simulink model "WaveStar"  (R2020b)
settings: Solver=ode8  StartTime=0  StopTime=225  FixedStep=0.05  MaxStep=0.05  RelTol=1e-3  EnableMultiTasking=on
values from neighbouring files (symbols this model uses):
  Ad = sysD.A    [controller_init.m]
  alpha_eff = ( eta_motoring + eta_generator ) / 2    (= 1.06428571429)    [controller_init.m]
  ARorder = 18    [controller_init.m]
  ARtrainingSet = 10    [controller_init.m]
  Bd = sysD.B    [controller_init.m]
  beta_eff = ( eta_motoring - eta_generator ) / 2    (= 0.364285714286)    [controller_init.m]
  dt = simu.dt    [controller_init.m]
  eta_generator = 0.7    [controller_init.m]
  eta_motoring = 1 / 0.7    (= 1.42857142857)    [controller_init.m]
  excM_precalculated = excM_stored    [controller_init.m]
  L_AB = 0.412    [controller_init.m]
  L_AC = 0.2    [controller_init.m]
  LAfloat = 0.54875    [controller_init.m]
  McSat = 12    [controller_init.m]
  Np = 40    [controller_init.m]
  phi_eff = 1000    [controller_init.m]
  predictionType = 2    [controller_init.m]
  prop_gain = 19.40;  load('waveData/SS6_excM_stored.mat')    [controller_init.m]
  Qkf = blkdiag( Qp, Qv, QradM, QexcM )    [controller_init.m]
  qnl = [ 0, 1; 1, 0 ]    [controller_init.m]
  R_ctrl = 0.90*eye( Np*nu )    [controller_init.m]
  Rkf = blkdiag( Rp, Rv )    [controller_init.m]
  startController = 15    [controller_init.m]
  startPredictor = 10    [controller_init.m]
  Theta0 = deg2rad(26.9527)    [controller_init.m]
  Umax = McSat    (= 12)    [controller_init.m]
  Umin = -McSat    (= -12)    [controller_init.m]
  xPcTs = dt    [controller_init.m]
undefined symbols (not defined in the file or in its folder): body, constraint, geometry, HPfreq, hydroData, LPfreq, pto, X, Y, Z
libraries: nesl_utility x9, WECSim_Lib_Constraints x5, WECSim_Lib_Body_Elements x5, sm_lib x5, WECSim_Lib_Frames x1
settings Model: Creator=kmruehl  LastModifiedBy=akeeste
settings SolverCC: ZeroCrossControl=DisableAll  AutoInsertRateTranBlk=on
settings DataIOCC: ReturnWorkspaceOutputs=off
settings OptimizationCC: LifeSpan=inf  SimCompilerOptimization=on
settings DebuggingCC: SFUnexpectedBacktrackingDiag=warning  SFNoUnconditionalDefaultTransitionDiag=warning  SFExecutionAtInitializationDiag=none  ArithmeticOperatorsInVariantConditions=warning
settings ModelReferenceCC: ModelReferenceMinAlgLoopOccurrences=on
settings SFSimCC: SimUseLocalCustomCode=off  CustomCodeUndefinedFunction=UseInterfaceOnly
settings RTWCC: RTWUseLocalCustomCode=off
settings CodeAppCC: StateflowObjectComments=on
settings GRTTargetCC: TargetLangStandard=C89/C90 (ANSI)
settings ConfigComp: CovMetricSettings=dw  CovSaveCumulativeToWorkspaceVar=on  CovSaveSingleToWorkspaceVar=on  CovExternalEMLEnable=off
settings SimscapeCC: SimscapeNormalizeSystem=off
settings ExplorerConfigSet: SimMechanicsOpenEditorOnUpdate=off  InternalSimMechanicsExplorerSettings="<ExplorerConfiguration><canonicalview>default</canonicalview><AnimationSetting><BasePlaybackSpeed>1.0</BasePlaybackSpeed><PlaybackSpeedFactor>1.0</PlaybackSpeedFactor></AnimationSetting><TilePanel><TileInfo><Tiles Columns=\"2\" Count=\"4\" Rows=\"2\"><Column Left=\"2\" Weight=\"0.4998\"/><Column Left=\"667\" Weight=\"0.5002\"/><Column Left=\"1333\"/><Row Top=\"2\" Weight=\"0.4997\"/><Row Top=\"952\" Weight=\"0.5003\"/><Row Top=\"1904\"/><Tile Height=\"1\" Width=\"1\" X=\"0\" Y=\"0\"/><Tile Height=\"1\" Width=\"1\" X=\"0\" Y=\"1\"/><Tile Height=\"1\" Width=\"1\" X=\"1\" Y=\"0\"/><Tile Height=\"1\" Width=\"1\" X=\"1\" Y=\"1\"/></Tiles></TileInfo><SceneInfo><SceneViewer><BGColor><R>0.60000002384185791</R><G>0.60000002384185791</G><B>0.60000002384185791</B></BGColor><Camera><DoPerspective>off</DoPerspective><Position><X>0.12470049519875293</X><Y>-7.8483064192972183</Y><Z>0.41049948909937695</Z></Position><Center><X>0.12470049519875293</X><Y>2.8810501090381635e-07</Y><Z>0.41049948909937695</Z></Center><Up><X>0</X><Y>-0</Y><Z>1</Z></Up><ViewLimDist>1</ViewLimDist><YLim>1.4359338132666335</YLim><XLim>1.0010335616396511</XLim></Camera></SceneViewer><SceneViewer><BGColor><R>0.60000002384185791</R><G>0.60000002384185791</G><B>0.60000002384185791</B></BGColor><Camera><DoPerspective>off</DoPerspective><Position><X>0.32732511337828807</X><Y>-0.082581165896399134</Y><Z>7.1171098135796953</Z></Position><Center><X>0.32732511337828807</X><Y>-0.082581165896399134</Y><Z>0.45174407037336595</Z></Center><Up><X>0</X><Y>1</Y><Z>-0</Z></Up><ViewLimDist>1</ViewLimDist><YLim>1.40160176353799</YLim><XLim>0.97502731376555829</XLim></Camera></SceneViewer><SceneViewer><BGColor><R>0.60000002384185791</R><G>0.60000002384185791</G><B>0.60000002384185791</B></BGColor><Camera><DoPerspective>off</DoPerspective><Position><X>7.848306419447999</X><Y>0.086028706913199554</Y><Z>0.42305679091343457</Z></Position><Center><X>-3.0318302890464111e-07</X><Y>0.086028706913199554</Y><Z>0.42305679091343457</Z></Center><Up><X>-0</X><Y>0</Y><Z>1</Z></Up><ViewLimDist>1</ViewLimDist><YLim>1.4671457032424258</YLim><XLim>1.0243514633690476</XLim></Camera></SceneViewer><SceneViewer><BGColor><R>0.60000002384185791</R><G>0.60000002384185791</G><B>0.60000002384185791</B></BGColor><Camera><DoPerspective>off</DoPerspective><Position><X>4.3109367218514292</X><Y>-3.7387044463777657</Y><Z>4.7725637716535374</Z></Position><Center><X>-0.21521500504762375</X><Y>0.78744728052128776</Y><Z>0.24641204475448614</Z></Center><Up><X>-0.40824829046386307</X><Y>0.40824829046386307</Y><Z>0.81649658092772615</Z></Up><ViewLimDist>1</ViewLimDist><YLim>1.979107791195027</YLim><XLim>1.3788693730807347</XLim></Camera></SceneViewer></SceneInfo></TilePanel><MechEditorPanel><Cameras/><GfxPanelCameraMap/><VideoCreator><PlaybackSpeedRatio>1.0</PlaybackSpeedRatio><FrameRate>30</FrameRate><VideoFormat>Motion JPEG AVI</VideoFormat><FrameSize>auto</FrameSize></VideoCreator></MechEditorPanel></ExplorerConfiguration>"

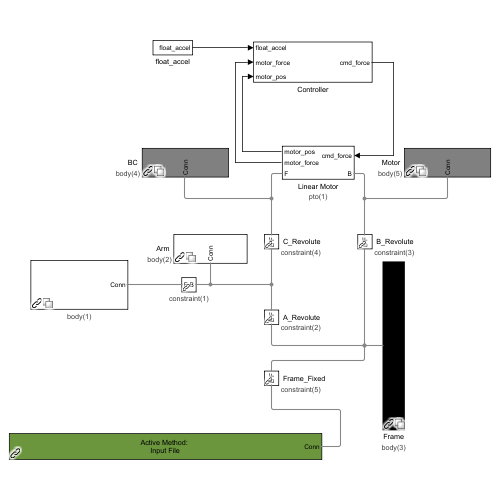
[thumbnail: Simulink's stored preview of the top-level diagram]
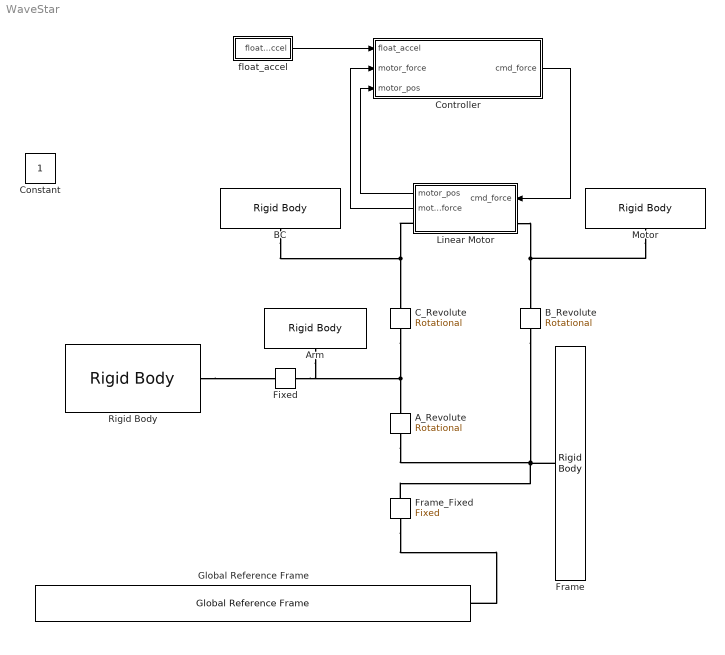
== system WaveStar ==
  A_Revolute : WECSim_Lib_Constraints/Rotational  constraint=constraint(2)  loc="-0.438           0       0.302"  displacement=0 0 0  y="0  1  0"  z="0  0  1"  upperLimitSpecify=off  upperLimitBound=1  upperLimitTransitionRegionWidth=0.0001  upperLimitStiffness=1000000  upperLimitDamping=1000  lowerLimitSpecify=off  lowerLimitBound=-1  lowerLimitTransitionRegionWidth=0.0001  lowerLimitStiffness=1000000  lowerLimitDamping=1000
      settings: AttributesFormatString=%<constraint>
  Arm : WECSim_Lib_Body_Elements/Rigid Body  body=body(2)  h5File=hydroData/*.h5  geometryFile=geometry/Arm.stl  mass=1.157  inertia=0 0 0  inertiaProducts=0 0 0  nonHydro=0  nonlinearHydro=0  centerGravity=0 0 0  centerBuoyancy=0 0 0  dof=6  volume=0  QTFs=0  displacement=0 0 0  axis=0 1 0  angle=0  option=0  cd="0  0  0"  ca="0  0  0"  area=0 0 0  VME=0  rgME="0  0  0"  z="0  0  1"
  BC : WECSim_Lib_Body_Elements/Rigid Body  body=body(4)  h5File=hydroData/*.h5  geometryFile=geometry/BC.stl  mass=0.0001  inertia=0 0 0  inertiaProducts=0 0 0  nonHydro=0  nonlinearHydro=0  centerGravity=0 0 0  centerBuoyancy=0 0 0  dof=6  volume=0  QTFs=0  displacement=0 0 0  axis=0 1 0  angle=0  option=0  cd="0  0  0"  ca="0  0  0"  area=0 0 0  VME=0  rgME="0  0  0"  z="0  0  1"
  B_Revolute : WECSim_Lib_Constraints/Rotational  constraint=constraint(3)  loc="-0.438           0       0.714"  displacement=0 0 0  y="0  1  0"  z="0  0  1"  upperLimitSpecify=off  upperLimitBound=1  upperLimitTransitionRegionWidth=0.0001  upperLimitStiffness=1000000  upperLimitDamping=1000  lowerLimitSpecify=off  lowerLimitBound=-1  lowerLimitTransitionRegionWidth=0.0001  lowerLimitStiffness=1000000  lowerLimitDamping=1000
      settings: AttributesFormatString=%<constraint>
  C_Revolute : WECSim_Lib_Constraints/Rotational  constraint=constraint(4)  loc="-0.62144           0     0.38169"  displacement=0 0 0  y="0  1  0"  z="0  0  1"  upperLimitSpecify=off  upperLimitBound=1  upperLimitTransitionRegionWidth=0.0001  upperLimitStiffness=1000000  upperLimitDamping=1000  lowerLimitSpecify=off  lowerLimitBound=-1  lowerLimitTransitionRegionWidth=0.0001  lowerLimitStiffness=1000000  lowerLimitDamping=1000
      settings: AttributesFormatString=%<constraint>
  Controller : Subsystem
  Fixed : WECSim_Lib_Constraints/Fixed  constraint=constraint(1)  loc="0           0        0.09"  displacement=0 0 0  y="0  1  0"  z="0  0  1"  upperLimitSpecify=off  upperLimitBound=1  upperLimitTransitionRegionWidth=0.0001  upperLimitStiffness=1000000  upperLimitDamping=1000  lowerLimitSpecify=off  lowerLimitBound=-1  lowerLimitTransitionRegionWidth=0.0001  lowerLimitStiffness=1000000  lowerLimitDamping=1000
      settings: AttributesFormatString=%<constraint>
  Frame : WECSim_Lib_Body_Elements/Rigid Body  body=body(3)  h5File=hydroData/*.h5  geometryFile=geometry/Frame.stl  mass=999  inertia=0 0 0  inertiaProducts=0 0 0  nonHydro=0  nonlinearHydro=0  centerGravity=0 0 0  centerBuoyancy=0 0 0  dof=6  volume=0  QTFs=0  displacement=0 0 0  axis=0 1 0  angle=0  option=0  cd="0  0  0"  ca="0  0  0"  area=0 0 0  VME=0  rgME="0  0  0"  z="0  0  1"
  Frame_Fixed : WECSim_Lib_Constraints/Fixed  constraint=constraint(5)  loc="-0.438           0         1.5"  displacement=0 0 0  y="0  1  0"  z="0  0  1"  upperLimitSpecify=off  upperLimitBound=1  upperLimitTransitionRegionWidth=0.0001  upperLimitStiffness=1000000  upperLimitDamping=1000  lowerLimitSpecify=off  lowerLimitBound=-1  lowerLimitTransitionRegionWidth=0.0001  lowerLimitStiffness=1000000  lowerLimitDamping=1000
      settings: AttributesFormatString=%<constraint>
  Global Reference Frame : WECSim_Lib_Frames/Global Reference Frame  waves=waves  simu=simu  InputMethod=Input File  InputFile=wecSimInputFile.m  mode=normal  explorer=off  solver=ode4  startTime=0  rampTime=25  endTime=200  dt=0.01  cicEndTime=60  stateSpace=0  WaveClass=etaImport  height=2.5  period=8  elevationFile=NOT DEFINED  spectrumFile=NOT DEFINED  direction=0  spread=1  spectrumType=NOT DEFINED  phaseSeed=0  option=EqualEnergy
  Linear Motor : Subsystem  mask(PTO){pto=pto(1)}
      mask prompts: pto "PTO Name:"
      mask help:
      | Constraints the follower to translational motion relative to the base, in
      | the PTO's Z-direction and adds PTO stiffness and damping. Also applies a
      | user-defined force and outputs extension, velocity, and acceleration.
      |
      |
      | The variable name input below must be 'pto(i)' where i=1,2,...
      | pto(i) must be defined in the input file with the following fields:
      |
      |     .name (required)
      |             String.
      |             PTO name. Must comply with Matlab's variable naming rules.
      |     .loc (optional)
      |             3x1 vector [x y z] in meters.
      |             PTO location. Default = [0 0 0]
      |     .k (optional)
      |             Float.
      |             PTO linear spring stiffness. Default = 0
      |     .c (optional)
      |             Float.
      |             PTO linear damping coefficient. Default = 0
      |     .orientation.z (optional)
      |             3x1 vector [x y z].
      |             Direction of the PTO's Z-coordinate. Default = [0 0 1]
      |     .orientation.y (optional)
      |             3x1 vector [x y z].
      |             Direction of the PTO's Y-coordinate. Default = [0 1 0]
      mask init:
      | if exist('pto','var')
      |     h=[gcb '/output'];
      |     responseName=['pto' num2str(pto.number) '_out'];
      |     set_param(h,'VariableName',responseName);
      | end
      | 
      | pto.checkLoc('W');
      settings: AttributesFormatString=%<pto>
      mask Help:
      | Constraints the follower to translational motion relative to the base, in
      | the PTO's Z-direction and adds PTO stiffness and damping. Also applies a
      | user-defined force and outputs extension, velocity, and acceleration.
      | 
      | 
      | The variable name input below must be 'pto(i)' where i=1,2,...
      | pto(i) must be defined in the input file with the following fields:
      | 
      |     .name (required)
      |             String.
      |             PTO name. Must comply with Matlab's variable naming rules.
      |     .loc (optional)
      |             3x1 vector [x y z] in meters.
      |             PTO location. Default = [0 0 0]
      |     .k (optional)
      |             Float.
      |             PTO linear spring stiffness. Default = 0
      |     .c (optional)
      |             Float.
      |             PTO linear damping coefficient. Default = 0
      |     .orientation.z (optional)
      |             3x1 vector [x y z].
      |             Direction of the PTO's Z-coordinate. Default = [0 0 1]
      |     .orientation.y (optional)
      |             3x1 vector [x y z].
      |             Direction of the PTO's Y-coordinate. Default = [0 1 0]
  Motor : WECSim_Lib_Body_Elements/Rigid Body  body=body(5)  h5File=hydroData/*.h5  geometryFile=geometry/Motor.stl  mass=0.0001  inertia=0 0 0  inertiaProducts=0 0 0  nonHydro=0  nonlinearHydro=0  centerGravity=0 0 0  centerBuoyancy=0 0 0  dof=6  volume=0  QTFs=0  displacement=0 0 0  axis=0 1 0  angle=0  option=0  cd="0  0  0"  ca="0  0  0"  area=0 0 0  VME=0  rgME="0  0  0"  z="0  0  1"
  Rigid Body : WECSim_Lib_Body_Elements/Rigid Body  body=body(1)  h5File=hydroData/*.h5  geometryFile=geometry/*.stl  mass=0  inertia=0 0 0  inertiaProducts=0 0 0  nonHydro=0  nonlinearHydro=0  centerGravity=0 0 0  centerBuoyancy=0 0 0  dof=6  volume=0  QTFs=0  displacement=0 0 0  axis=0 1 0  angle=0  option=0  cd=0 0 0  ca=0 0 0  area=0 0 0  VME=0  rgME=0 0 0  z=0 0 1
  float_accel : Subsystem
  Constant : Constant  IOType=siggen
  wires:
  Controller/1(cmd_force) -> Linear Motor/1(cmd_force)
  float_accel/1(float_accel) -> Controller/1(float_accel)
  Linear Motor/1(motor_pos) -> Controller/3("motor_pos ")
  Linear Motor/2(motor_force) -> Controller/2(motor_force)
  connections:
  A_Revolute/LConn1 -- Frame_Fixed/RConn1 -- Frame/RConn1 -- B_Revolute/LConn1
  Frame_Fixed/LConn1 -- Global Reference Frame/RConn1
  C_Revolute/LConn1 -- A_Revolute/RConn1 -- Fixed/LConn1 -- Arm/RConn1
  Linear Motor/RConn1 -- BC/RConn1 -- C_Revolute/RConn1
  Motor/RConn1 -- B_Revolute/RConn1 -- Linear Motor/LConn1
  Rigid Body/RConn1 -- Fixed/RConn1

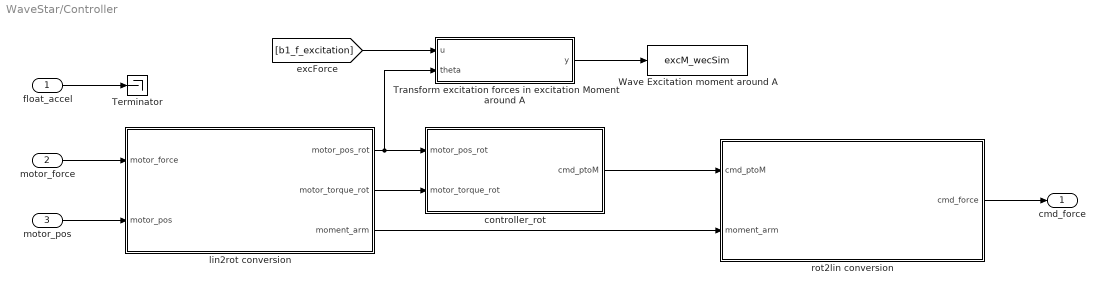
== system WaveStar/Controller ==
  float_accel : Inport
  motor_force : Inport  Port=2
  "motor_pos " : Inport  Port=3
  Terminator : Terminator
  Transform excitation forces in excitation Moment around A : MATLAB Function  TreatAsAtomicUnit=on
  Wave Excitation moment around A : ToWorkspace  VariableName=excM_wecSim  SaveFormat=Structure With Time  SampleTime=-1
  controller_rot : Subsystem
  lin2rot conversion : Subsystem
  rot2lin conversion : Subsystem
  cmd_force : Outport
  wires:
  Transform excitation forces in excitation Moment around A/1(y) -> Wave Excitation moment around A/1
  [b1_f_excitation] -> Transform excitation forces in excitation Moment around A/1(u)
  lin2rot conversion/1(motor_pos_rot) -> Transform excitation forces in excitation Moment around A/2(theta), controller_rot/1("motor_pos_rot ")
  motor_force/1 -> lin2rot conversion/1(motor_force)
  "motor_pos "/1 -> lin2rot conversion/2("motor_pos ")
  float_accel/1 -> Terminator/1
  rot2lin conversion/1(cmd_force) -> cmd_force/1
  lin2rot conversion/2(motor_torque_rot) -> controller_rot/2(motor_torque_rot)
  lin2rot conversion/3(moment_arm) -> rot2lin conversion/2(moment_arm)
  controller_rot/1(cmd_ptoM) -> rot2lin conversion/1(cmd_ptoM)

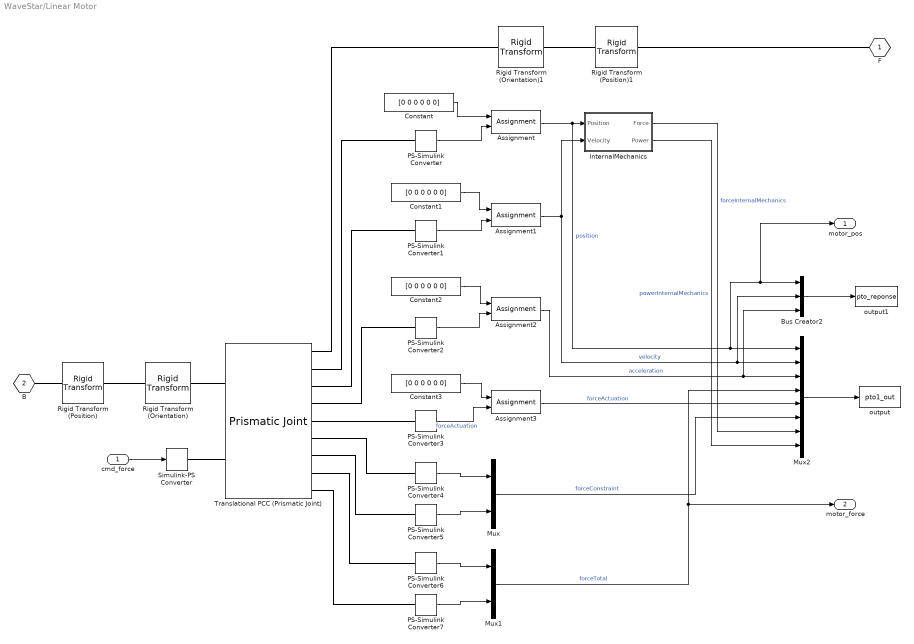
== system WaveStar/Linear Motor ==
  cmd_force : Inport
  Assignment{,1..3} (4 alike) : Assignment  IndexOptions=Index vector (dialog)  Indices=3  OutputSizes=1
  Bus Creator2 : BusCreator  Inputs=3
  Constant{,1..3} (4 alike) : Constant  Value=[0 0 0 0 0 0]
  InternalMechanics : Subsystem
  Mux : Mux  Inputs=2
  Mux1 : Mux  Inputs=2
  Mux2 : Mux  Inputs=8
  PS-Simulink Converter{,1..7} (8 alike) : nesl_utility/PS-Simulink Converter  PhysicalDomain=network_engine_domain  SubClassName=ps_output  LeftPortType=input  RightPortType=output  PseudoPeriodic=off  Frequencies=[]  VectorFormat=1-D array  Unit=1  AffineConversion=off
  Rigid Transform (Position) : sm_lib/Frames and Transforms/Rigid Transform  RotationMethod=None  FollAlignAxisA=+X  BaseAlignAxisA=+Y  FollAlignAxisB=+Y  BaseAlignAxisB=+Z  RotationStandardAxis=+Y  RotationAngle=0  RotationAngleUnits=rad  RotationArbitraryAxis=[0 1 0]  RotationSequenceAxes=FollowerAxes  RotationSequence=XYX  RotationSequenceAngles=[0 0 0]  RotationSequenceAnglesUnits=deg  RotationMatrix=[1 0 0; 0 1 0; 0 0 1]  Quaternion=[1 0 0 0]  TranslationMethod=Cartesian  TranslationCartesianOffset=pto.initial.displacement + pto.location  TranslationCartesianOffsetUnits=m  TranslationStandardAxis=+Z  TranslationStandardOffset=0  TranslationStandardOffsetUnits=m  TranslationROffset=0  TranslationROffsetUnits=m  TranslationThetaOffset=0  TranslationThetaOffsetUnits=deg  TranslationZOffset=0  TranslationZOffsetUnits=m
  Rigid Transform (Position)1 : sm_lib/Frames and Transforms/Rigid Transform  RotationMethod=None  FollAlignAxisA=+X  BaseAlignAxisA=+Y  FollAlignAxisB=+Y  BaseAlignAxisB=+Z  RotationStandardAxis=+Y  RotationAngle=0  RotationAngleUnits=rad  RotationArbitraryAxis=[0 1 0]  RotationSequenceAxes=FollowerAxes  RotationSequence=XYX  RotationSequenceAngles=[0 0 0]  RotationSequenceAnglesUnits=deg  RotationMatrix=[1 0 0; 0 1 0; 0 0 1]  Quaternion=[1 0 0 0]  TranslationMethod=Cartesian  TranslationCartesianOffset=pto.initial.displacement + pto.location  TranslationCartesianOffsetUnits=m  TranslationStandardAxis=+Z  TranslationStandardOffset=0  TranslationStandardOffsetUnits=m  TranslationROffset=0  TranslationROffsetUnits=m  TranslationThetaOffset=0  TranslationThetaOffsetUnits=deg  TranslationZOffset=0  TranslationZOffsetUnits=m
  Rigid Transform (Orientation) : sm_lib/Frames and Transforms/Rigid Transform  RotationMethod=RotationMatrix  FollAlignAxisA=+X  BaseAlignAxisA=+Y  FollAlignAxisB=+Y  BaseAlignAxisB=+Z  RotationStandardAxis=+Y  RotationAngle=0  RotationAngleUnits=rad  RotationArbitraryAxis=[0 1 0]  RotationSequenceAxes=FollowerAxes  RotationSequence=XYX  RotationSequenceAngles=[0 0 0]  RotationSequenceAnglesUnits=deg  RotationMatrix=pto.orientation.rotationMatrix  Quaternion=[1 0 0 0]  TranslationMethod=None  TranslationCartesianOffset=0  TranslationCartesianOffsetUnits=m  TranslationStandardAxis=+Z  TranslationStandardOffset=0  TranslationStandardOffsetUnits=m  TranslationROffset=0  TranslationROffsetUnits=m  TranslationThetaOffset=0  TranslationThetaOffsetUnits=deg  TranslationZOffset=0  TranslationZOffsetUnits=m
  Rigid Transform (Orientation)1 : sm_lib/Frames and Transforms/Rigid Transform  RotationMethod=RotationMatrix  FollAlignAxisA=+X  BaseAlignAxisA=+Y  FollAlignAxisB=+Y  BaseAlignAxisB=+Z  RotationStandardAxis=+Y  RotationAngle=0  RotationAngleUnits=rad  RotationArbitraryAxis=[0 1 0]  RotationSequenceAxes=FollowerAxes  RotationSequence=XYX  RotationSequenceAngles=[0 0 0]  RotationSequenceAnglesUnits=deg  RotationMatrix=pto.orientation.rotationMatrix  Quaternion=[1 0 0 0]  TranslationMethod=None  TranslationCartesianOffset=0  TranslationCartesianOffsetUnits=m  TranslationStandardAxis=+Z  TranslationStandardOffset=0  TranslationStandardOffsetUnits=m  TranslationROffset=0  TranslationROffsetUnits=m  TranslationThetaOffset=0  TranslationThetaOffsetUnits=deg  TranslationZOffset=0  TranslationZOffsetUnits=m
  Simulink-PS Converter : nesl_utility/Simulink-PS Converter  PhysicalDomain=network_engine_domain  SubClassName=ps_input  LeftPortType=input  RightPortType=output  PseudoPeriodic=off  Frequencies=[]  NoiseDistribution=none  NoiseParameters=[]  Unit=1  AffineConversion=off  FilteringAndDerivatives=zero  SimscapeFilterOrder=1  InputFilterTimeConstant=0.001  UdotUserProvided=1
  Translational PCC (Prismatic Joint) : sm_lib/Joints/Prismatic Joint  JointMode=Normal  CompositeWrenchDir=BaseOnFollower  CompositeWrenchFrame=BaseFrame  SenseConstraintForce=on  SenseConstraintTorque=on  SenseTotalForce=on  SenseTotalTorque=on  PositionTargetSpecify=off  PositionTargetPriority=High  PositionTargetValue=0  PositionTargetValueUnits=m  VelocityTargetSpecify=off  VelocityTargetPriority=High  VelocityTargetValue=0  VelocityTargetValueUnits=m/s  EquilibriumPosition=0  EquilibriumPositionUnits=m  SpringStiffness=pto.stiffness  SpringStiffnessUnits=N/m  DampingCoefficient=pto.damping  DampingCoefficientUnits=N/(m/s)  LowerLimitSpecify=off  LowerLimitBound=-1  LowerLimitBoundUnits=m  LowerLimitStiffness=1e6  LowerLimitStiffnessUnits=N/m  LowerLimitDamping=1e3  LowerLimitDampingUnits=N/(m/s)  LowerLimitTransitionRegionWidth=1e-4  LowerLimitTransitionRegionWidthUnits=m  UpperLimitSpecify=off  UpperLimitBound=1  UpperLimitBoundUnits=m  UpperLimitStiffness=1e6  UpperLimitStiffnessUnits=N/m  UpperLimitDamping=1e3  UpperLimitDampingUnits=N/(m/s)  UpperLimitTransitionRegionWidth=1e-4  UpperLimitTransitionRegionWidthUnits=m  TorqueActuationMode=InputTorque  MotionActuationMode=ComputedMotion  SensePosition=on  SenseVelocity=on  SenseAcceleration=on  SenseTorqueForce=on  SenseLowerLimitTorqueForce=off  SenseUpperLimitTorqueForce=off
  output : ToWorkspace  VariableName=pto1_out  SaveFormat=Structure With Time  SampleTime=-1
      settings: Decimation=round(simu.dtOut/simu.dt,0)
  output1 : ToWorkspace  VariableName=pto_reponse  SaveFormat=Structure With Time  SampleTime=-1
      settings: Decimation=round(simu.dtOut/simu.dt,0)
  F : PMIOPort  Side=Right
  B : PMIOPort  Port=2  Side=Left
  motor_pos : Outport  VectorParamsAs1DForOutWhenUnconnected=off
  motor_force : Outport  Port=2  VectorParamsAs1DForOutWhenUnconnected=off
  wires:
  Assignment/1 -> Mux2/1, motor_pos/1, Bus Creator2/1, InternalMechanics/1(Position)  "position"
  Assignment1/1 -> Mux2/2, Bus Creator2/2, InternalMechanics/2(Velocity)  "velocity"
  Assignment2/1 -> Mux2/3, Bus Creator2/3  "acceleration"
  cmd_force/1 -> Simulink-PS Converter/1
  Mux2/1 -> output/1
  Mux/1 -> Mux2/6  "forceConstraint"
  Mux1/1 -> motor_force/1, Mux2/4  "forceTotal"
  PS-Simulink Converter4/1 -> Mux/1
  PS-Simulink Converter5/1 -> Mux/2
  PS-Simulink Converter6/1 -> Mux1/1
  PS-Simulink Converter7/1 -> Mux1/2
  Assignment3/1 -> Mux2/5  "forceActuation"
  Constant/1 -> Assignment/1
  PS-Simulink Converter/1 -> Assignment/2
  Constant1/1 -> Assignment1/1
  PS-Simulink Converter1/1 -> Assignment1/2
  Constant2/1 -> Assignment2/1
  PS-Simulink Converter2/1 -> Assignment2/2
  InternalMechanics/1(Force) -> Mux2/7  "forceInternalMechanics"
  InternalMechanics/2(Power) -> Mux2/8  "powerInternalMechanics"
  Constant3/1 -> Assignment3/1
  PS-Simulink Converter3/1 -> Assignment3/2  "forceActuation"
  Bus Creator2/1 -> output1/1
  connections:
  Rigid Transform (Position)/RConn1 -- Rigid Transform (Orientation)/LConn1
  Rigid Transform (Position)1/RConn1 -- Rigid Transform (Orientation)1/LConn1
  Simulink-PS Converter/RConn1 -- Translational PCC (Prismatic Joint)/LConn2
  Rigid Transform (Orientation)/RConn1 -- Translational PCC (Prismatic Joint)/LConn1
  Rigid Transform (Position)/LConn1 -- B/RConn1
  Translational PCC (Prismatic Joint)/RConn5 -- PS-Simulink Converter3/LConn1
  Translational PCC (Prismatic Joint)/RConn9 -- PS-Simulink Converter7/LConn1
  Rigid Transform (Orientation)1/RConn1 -- Translational PCC (Prismatic Joint)/RConn1
  Translational PCC (Prismatic Joint)/RConn4 -- PS-Simulink Converter2/LConn1
  Translational PCC (Prismatic Joint)/RConn7 -- PS-Simulink Converter5/LConn1
  Translational PCC (Prismatic Joint)/RConn3 -- PS-Simulink Converter1/LConn1
  Rigid Transform (Position)1/LConn1 -- F/RConn1
  Translational PCC (Prismatic Joint)/RConn8 -- PS-Simulink Converter6/LConn1
  Translational PCC (Prismatic Joint)/RConn2 -- PS-Simulink Converter/LConn1
  Translational PCC (Prismatic Joint)/RConn6 -- PS-Simulink Converter4/LConn1

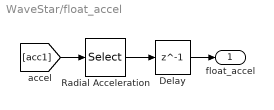
== system WaveStar/float_accel ==
  Delay : Delay  DelayLength=1  InitialCondition=0
  Radial Acceleration : Selector  InputPortWidth=6  IndexOptions=Index vector (dialog)  Indices=[5]  OutputSizes=1
  float_accel : Outport  VectorParamsAs1DForOutWhenUnconnected=off
  wires:
  [acc1] -> Radial Acceleration/1
  Radial Acceleration/1 -> Delay/1
  Delay/1 -> float_accel/1

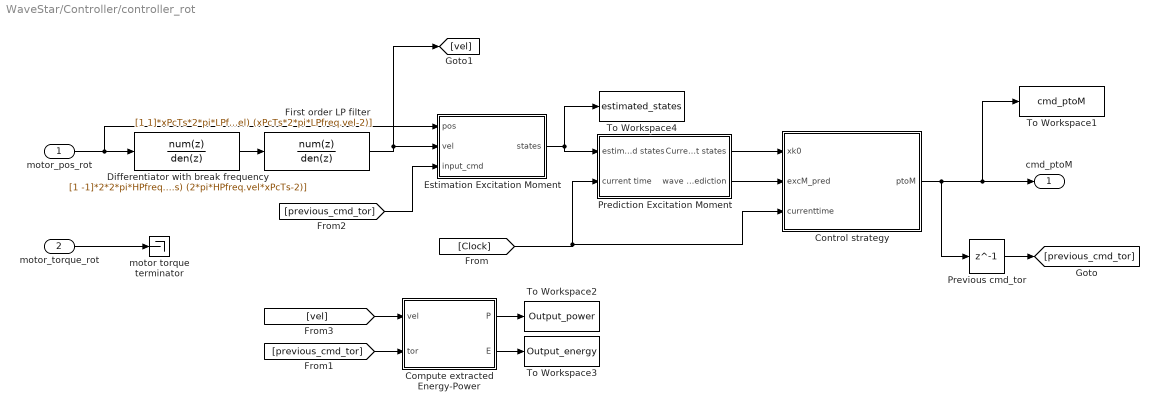
== system WaveStar/Controller/controller_rot ==
  "motor_pos_rot " : Inport
  motor_torque_rot : Inport  Port=2
  Compute extracted Energy-Power : MATLAB Function  TreatAsAtomicUnit=on
  Control strategy : Subsystem  Variant=on  VariantControl=Choice
  Differentiator with break frequency : DiscreteTransferFcn  Numerator=[1 -1]*2*2*pi*HPfreq.vel  Denominator=[(2+2*pi*HPfreq.vel*xPcTs) (2*pi*HPfreq.vel*xPcTs-2)]
  "Estimation Excitation Moment " : MATLAB Function  TreatAsAtomicUnit=on
  First order LP filter : DiscreteTransferFcn  Numerator=[1 1]*xPcTs*2*pi*LPfreq.vel  Denominator=[(2+xPcTs*2*pi*LPfreq.vel) (xPcTs*2*pi*LPfreq.vel-2)]
  "Prediction Excitation Moment " : Subsystem
  Previous cmd_tor : Delay  DelayLength=1
  To Workspace1 : ToWorkspace  VariableName=cmd_ptoM  SaveFormat=Structure With Time  SampleTime=-1
  To Workspace2 : ToWorkspace  VariableName=Output_power  SaveFormat=Structure With Time  SampleTime=-1
  To Workspace3 : ToWorkspace  VariableName=Output_energy  SaveFormat=Structure With Time  SampleTime=-1
  To Workspace4 : ToWorkspace  VariableName=estimated_states  SaveFormat=Structure With Time  SampleTime=-1
  motor torque terminator : Terminator
  cmd_ptoM : Outport  VectorParamsAs1DForOutWhenUnconnected=off
  wires:
  Differentiator with break frequency/1 -> First order LP filter/1
  motor_torque_rot/1 -> motor torque terminator/1
  "motor_pos_rot "/1 -> "Estimation Excitation Moment "/1(pos), Differentiator with break frequency/1
  First order LP filter/1 -> [vel], "Estimation Excitation Moment "/2(vel)
  "Estimation Excitation Moment "/1(states) -> "Prediction Excitation Moment "/1(estimated states), To Workspace4/1
  Compute extracted Energy-Power/1(P) -> To Workspace2/1
  Compute extracted Energy-Power/2(E) -> To Workspace3/1
  Control strategy/1(ptoM) -> Previous cmd_tor/1, To Workspace1/1, cmd_ptoM/1
  "Prediction Excitation Moment "/1(Current states) -> Control strategy/1(xk0)
  "Prediction Excitation Moment "/2(wave prediction) -> Control strategy/2(excM_pred)
  [Clock] -> "Prediction Excitation Moment "/2(current time), Control strategy/3(currenttime)
  Previous cmd_tor/1 -> [previous_cmd_tor]
  [previous_cmd_tor] -> "Estimation Excitation Moment "/3(input_cmd)
  [previous_cmd_tor] -> Compute extracted Energy-Power/2(tor)
  [vel] -> Compute extracted Energy-Power/1(vel)

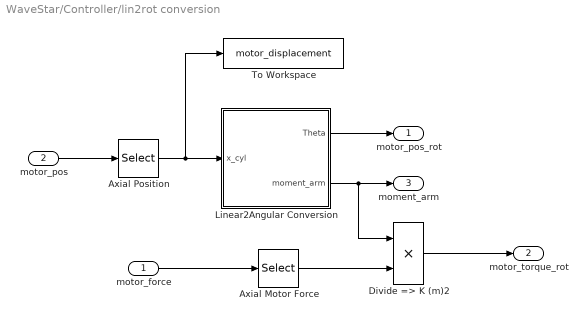
== system WaveStar/Controller/lin2rot conversion ==
  motor_force : Inport
  "motor_pos " : Inport  Port=2
  Axial Motor Force : Selector  InputPortWidth=6  IndexOptions=Index vector (dialog)  Indices=[3]  OutputSizes=1
  Axial Position : Selector  InputPortWidth=6  IndexOptions=Index vector (dialog)  Indices=[3]  OutputSizes=1
  Divide => K (m)2 : Product  Inputs=**
  Linear2Angular Conversion : Subsystem
  To Workspace : ToWorkspace  VariableName=motor_displacement  SaveFormat=Structure With Time  SampleTime=-1
  motor_pos_rot : Outport  VectorParamsAs1DForOutWhenUnconnected=off
  motor_torque_rot : Outport  Port=2  VectorParamsAs1DForOutWhenUnconnected=off
  moment_arm : Outport  Port=3  VectorParamsAs1DForOutWhenUnconnected=off
  wires:
  Linear2Angular Conversion/1(Theta) -> motor_pos_rot/1
  Divide => K (m)2/1 -> motor_torque_rot/1
  "motor_pos "/1 -> Axial Position/1
  Axial Position/1 -> To Workspace/1, Linear2Angular Conversion/1(x_cyl)
  motor_force/1 -> Axial Motor Force/1
  Axial Motor Force/1 -> Divide => K (m)2/2
  Linear2Angular Conversion/2(moment_arm) -> Divide => K (m)2/1, moment_arm/1

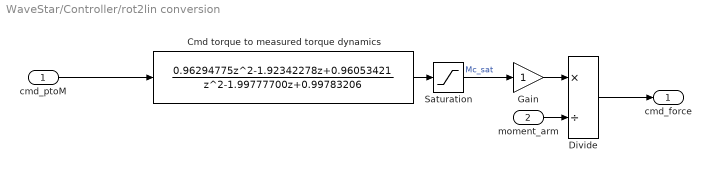
== system WaveStar/Controller/rot2lin conversion ==
  cmd_ptoM : Inport
  moment_arm : Inport  Port=2
  Cmd torque to measured torque dynamics : DiscreteTransferFcn  Numerator="[0.96294775   -1.92342278    0.96053421]"  Denominator="[1.00000000   -1.99777700    0.99783206]"
  "Divide " : Product  Inputs=*/
  Gain : Gain
  Saturation : Saturate  UpperLimit=McSat  LowerLimit=-McSat
  cmd_force : Outport  VectorParamsAs1DForOutWhenUnconnected=off
  wires:
  "Divide "/1 -> cmd_force/1
  moment_arm/1 -> "Divide "/2
  Saturation/1 -> Gain/1  "Mc_sat"
  Gain/1 -> "Divide "/1
  cmd_ptoM/1 -> Cmd torque to measured torque dynamics/1
  Cmd torque to measured torque dynamics/1 -> Saturation/1

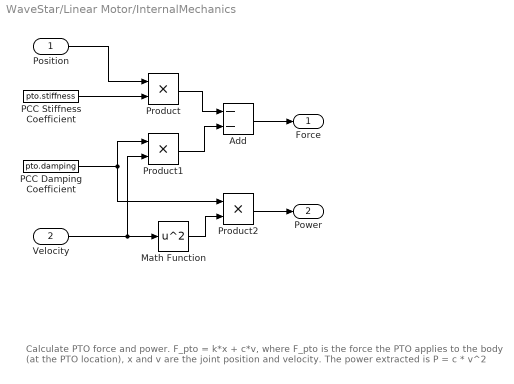
== system WaveStar/Linear Motor/InternalMechanics ==
  note: Calculate PTO force and power.
      |
      | F_pto  = k*x + c*v,
      | where F_pto is the force the PTO applies to the body (at the PTO location), x and v are the joint position and velocity.
      |
      | The power extracted is
      | P = c * v^2
  Position : Inport
  Velocity : Inport  Port=2
  Add : Sum  Inputs=--
  Math Function : Math  Operator=square  SignedPower=on  SaturateOnIntegerOverflow=on
  PCC Damping Coefficient : Constant  Value=pto.damping
  PCC Stiffness Coefficient : Constant  Value=pto.stiffness
  Product : Product  Inputs=**
  Product1 : Product  Inputs=**
  Product2 : Product  Inputs=**
  Force : Outport  VectorParamsAs1DForOutWhenUnconnected=off
  Power : Outport  Port=2  VectorParamsAs1DForOutWhenUnconnected=off
  wires:
  PCC Damping Coefficient/1 -> Product2/1, Product1/1
  Product2/1 -> Power/1
  Velocity/1 -> Math Function/1, Product1/2
  PCC Stiffness Coefficient/1 -> Product/2
  Position/1 -> Product/1
  Add/1 -> Force/1
  Math Function/1 -> Product2/2
  Product/1 -> Add/1
  Product1/1 -> Add/2

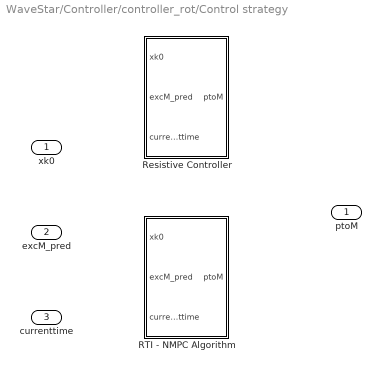
== system WaveStar/Controller/controller_rot/Control strategy ==
  xk0 : Inport
  excM_pred : Inport  Port=2
  currenttime : Inport  Port=3
  RTI - NMPC Algorithm : MATLAB Function  TreatAsAtomicUnit=on  VariantControl=controllerType == 2
  Resistive Controller : MATLAB Function  TreatAsAtomicUnit=on  VariantControl=controllerType == 1
  ptoM : Outport

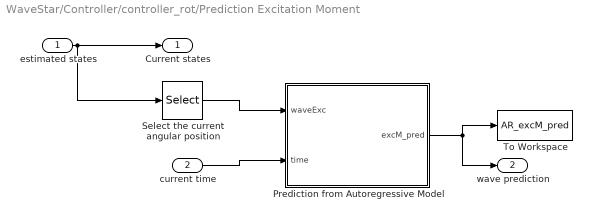
== system WaveStar/Controller/controller_rot/Prediction Excitation Moment  ==
  estimated states : Inport
  current time : Inport  Port=2
  "Prediction from Autoregressive Model " : MATLAB Function  TreatAsAtomicUnit=on
  Select the current angular position : Selector  InputPortWidth=5  IndexOptions=Index vector (dialog)  Indices=5  OutputSizes=1
  To Workspace : ToWorkspace  VariableName=AR_excM_pred  SaveFormat=Structure With Time  SampleTime=-1
  Current states : Outport
  wave prediction : Outport  Port=2
  wires:
  current time/1 -> "Prediction from Autoregressive Model "/2(time)
  Select the current angular position/1 -> "Prediction from Autoregressive Model "/1(waveExc)
  "Prediction from Autoregressive Model "/1(excM_pred) -> To Workspace/1, wave prediction/1
  estimated states/1 -> Select the current angular position/1, Current states/1

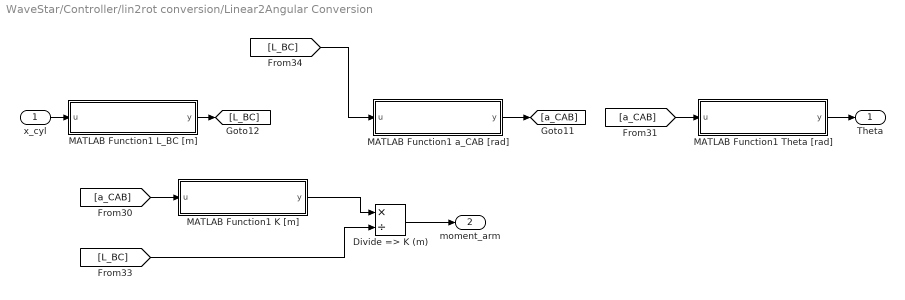
== system WaveStar/Controller/lin2rot conversion/Linear2Angular Conversion ==
  x_cyl : Inport
  Divide => K (m) : Product  Inputs=*/
  MATLAB Function1 K [m] : MATLAB Function  TreatAsAtomicUnit=on
  MATLAB Function1 L_BC [m] : MATLAB Function  TreatAsAtomicUnit=on
  MATLAB Function1 Theta [rad] : MATLAB Function  TreatAsAtomicUnit=on
  MATLAB Function1 a_CAB [rad] : MATLAB Function  TreatAsAtomicUnit=on
  Theta : Outport  VectorParamsAs1DForOutWhenUnconnected=off
  moment_arm : Outport  Port=2  VectorParamsAs1DForOutWhenUnconnected=off
  wires:
  MATLAB Function1 L_BC [m]/1(y) -> [L_BC]
  [a_CAB] -> MATLAB Function1 Theta [rad]/1(u)
  MATLAB Function1 K [m]/1(y) -> Divide => K (m)/1
  [L_BC] -> MATLAB Function1 a_CAB [rad]/1(u)
  [L_BC] -> Divide => K (m)/2
  x_cyl/1 -> MATLAB Function1 L_BC [m]/1(u)
  Divide => K (m)/1 -> moment_arm/1
  MATLAB Function1 a_CAB [rad]/1(y) -> [a_CAB]
  [a_CAB] -> MATLAB Function1 K [m]/1(u)
  MATLAB Function1 Theta [rad]/1(y) -> Theta/1

== matlab function WaveStar/Controller/controller_rot/Control strategy/RTI - NMPC Algorithm ==
  settings: updateMethod=DISCRETE
  data: xk0 input; ptoM output size=1; excM_pred input size=[Np,1]; Ad parameter; Bd parameter; R_ctrl parameter; Np parameter size=1; alpha_eff parameter size=1; beta_eff parameter size=1; phi_eff parameter size=1; qnl parameter; Umax parameter size=1; Umin parameter size=1; currenttime input size=1; startController parameter size=1; prop_gain parameter size=1
function ptoM = RTI_NMPC(xk0, excM_pred, Ad, Bd, R_ctrl, Np, alpha_eff, beta_eff, phi_eff, qnl, Umax, Umin,currenttime, startController, prop_gain)
    coder.extrinsic('NMPC');
    %Augmented system to include the previous control input in the state vector
    A   = blkdiag( Ad, 0 );                          %Augmented State Transition Matrix
    Bw  = [ Bd;  0 ];                                %Augmented Wave Input Matrix
    Bu  = [ Bd;  1 ];                                %Augmented Input Matrix
    Ubar = zeros(Np,1);
    if (currenttime >= 10) && (currenttime < startController)
       ptoM = - prop_gain * xk0(2);
    elseif (currenttime >= startController)
       Ubar = NMPC( xk0, excM_pred, A, Bu, Bw, R_ctrl, Np, alpha_eff, beta_eff, phi_eff, qnl, Umax, Umin);
       ptoM = Ubar(1,1);
    else
        ptoM = 0;
    end
    

   if ptoM >= Umax
       ptoM = Umax;
   elseif ptoM <= Umin
       ptoM = Umin;
   end

== matlab function WaveStar/Controller/controller_rot/Compute extracted Energy-Power ==
  data: vel input; P output; tor input; E output; eta_generator parameter; eta_motoring parameter; dt parameter
function [P, E] = Power(vel,tor, eta_generator, eta_motoring, dt)
                
    [P, E] = extractedPower(vel,tor, eta_generator, eta_motoring, dt);

== matlab function WaveStar/Controller/controller_rot/Control strategy/Resistive Controller ==
  settings: updateMethod=DISCRETE
  data: xk0 input; ptoM output size=1; excM_pred input size=[Np,1]; Umax parameter size=1; Umin parameter size=1; currenttime input size=1; startController parameter size=1; prop_gain parameter size=1
function ptoM = resistive(xk0, excM_pred, Umax, Umin,currenttime, startController, prop_gain)

    if currenttime >= startController
       ptoM = - prop_gain * xk0(2);
           if ptoM >= Umax
               ptoM = Umax;
           elseif ptoM<=Umin
               ptoM = Umin;
           end
    else
        ptoM = 0*excM_pred(1);
    end

== matlab function WaveStar/Controller/lin2rot conversion/Linear2Angular Conversion/MATLAB Function1 K [m] ==
  data: u input; y output; L_AB parameter; L_AC parameter
function y = fcn(u,L_AB,L_AC)
%#codegen
y = L_AB'*L_AC'*sin(u);

== matlab function WaveStar/Controller/lin2rot conversion/Linear2Angular Conversion/MATLAB Function1 L_BC [m] ==
  data: u input; y output; L_BC_neutral parameter
 function y = fcn(u,L_BC_neutral)
%#codegen
%
y = u+L_BC_neutral';

== matlab function WaveStar/Controller/lin2rot conversion/Linear2Angular Conversion/MATLAB Function1 Theta [rad] ==
  data: u input; y output; a_CAB_neutral parameter
function y = fcn(u,a_CAB_neutral)
%#codegen
y = u-a_CAB_neutral';

== matlab function WaveStar/Controller/Transform excitation forces in excitation Moment around A ==
  data: u input; theta input size=1; y output size=1; LAfloat parameter size=1; Theta0 parameter size=1
function y = transfExcMoment( u, theta, LAfloat, Theta0)

xFexc       = u( 1 );
zFexc       = u( 3 );
pitchMexc   = u( 5 );

y = (-LAfloat * xFexc .*sin( Theta0 + theta ) - zFexc * LAfloat.*cos( Theta0 + theta ) + pitchMexc );

== matlab function WaveStar/Controller/lin2rot conversion/Linear2Angular Conversion/MATLAB Function1 a_CAB [rad] ==
  data: u input; y output; L_AB parameter; L_AC parameter
function y = fcn(u,L_AB,L_AC)
%#codegen
%
y = acos((u.^2-L_AB'^2-L_AC'^2)/(-2*L_AB'*L_AC'));

== matlab function WaveStar/Controller/controller_rot/Estimation Excitation Moment  ==
  settings: updateMethod=DISCRETE
  data: pos input; vel input; input_cmd input; states output; Ad parameter; Bd parameter; Qkf parameter; Rkf parameter
function states = observer(pos, vel, input_cmd,  Ad, Bd, Qkf, Rkf)
                       
    u = [pos;
         vel];

states = observer_kf(input_cmd, u, Ad, Bd, Qkf, Rkf);

== matlab function WaveStar/Controller/controller_rot/Prediction Excitation Moment /Prediction from Autoregressive Model  ==
  settings: updateMethod=DISCRETE
  data: waveExc input size=1; Np parameter size=1; ARorder parameter size=1; time input size=1; startPredictor parameter size=1; excM_pred output size=[Np, 1]; ARtrainingSet parameter size=1; dt parameter; excM_precalculated parameter; predictionType parameter
function excM_pred =  vectorExcMpred(waveExc, Np, ARorder, time, startPredictor, ARtrainingSet, dt, excM_precalculated, predictionType)
    coder.extrinsic('predictor');

    persistent past_excM
    if isempty(past_excM)
        past_excM = zeros( ARtrainingSet*ARorder, 1 );
    end

    past_excM = [past_excM(2:end,1); waveExc];
    excM_pred   = zeros(Np,1);
   
    if time >= startPredictor
        switch(predictionType)
        % 1 to use the precalculated excM obtained from wecSim.
        % 2 to use the excM prediction from the AR algorithm.
            case 1
                  currentTime_index = uint64( time / dt );
                  excM_pred  = excM_precalculated(currentTime_index + 1 : currentTime_index + Np );
            case 2
                  excM_pred  = predictor(past_excM, ARorder, Np, time);
         end 
    end
